simulink model "P3_model"  (R2025b)
settings: Solver=ode4  StartTime=0.0  StopTime=3  FixedStep=20e-6  RelTol=1e-3
model workspace (MATLAB code in the model file):
  | J = 0.01;  B = 0.10;                 % 참 플랜트
  | Jm = 0.01; Bm = 0.03;                % 공칭 모델
  | lam = 40;  Ts = 1e-3;  umax = 2;
  | beta = 0.37; phi = 0.05;             % phi = 0 이면 sgn
  | k = 1e-3;  rho = 0;  wc = 100;
  | adapt_on = 0; dob_on = 0;
  | dz = 0; vel_diff = 0; sigma_x = 0;   % 보너스용
  | P = struct('Jm',Jm,'Bm',Bm,'lam',lam,'Ts',Ts,'umax',umax, ...
  |            'beta',beta,'phi',phi,'k',k,'rho',rho,'wc',wc, ...
  |            'adapt_on',adapt_on,'dob_on',dob_on,'dz',dz,'vel_diff',vel_diff);
settings Model: Creator=Owner  LastModifiedBy=Owner

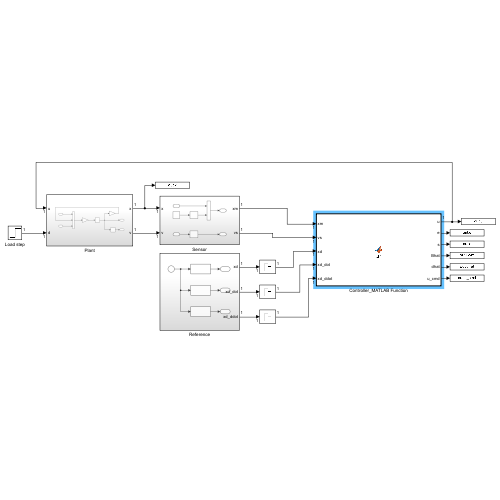
[thumbnail: Simulink's stored preview of the top-level diagram]
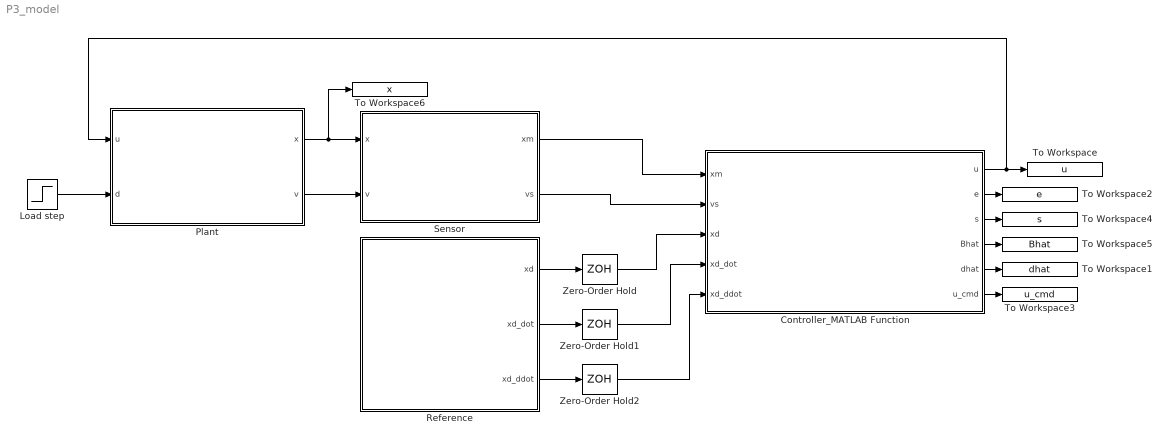
== system P3_model ==
  Controller_MATLAB Function : MATLAB Function  TreatAsAtomicUnit=on
  Load step : Step  Time=1.5  After=0.1  SampleTime=0
  Plant : Subsystem
  Reference : Subsystem
  Sensor : Subsystem
  To Workspace : ToWorkspace  VariableName=u  SaveFormat=Timeseries  SampleTime=-1
  To Workspace1 : ToWorkspace  VariableName=dhat  SaveFormat=Timeseries  SampleTime=-1
  To Workspace2 : ToWorkspace  VariableName=e  SaveFormat=Timeseries  SampleTime=-1
  To Workspace3 : ToWorkspace  VariableName=u_cmd  SaveFormat=Timeseries  SampleTime=-1
  To Workspace4 : ToWorkspace  VariableName=s  SaveFormat=Timeseries  SampleTime=-1
  To Workspace5 : ToWorkspace  VariableName=Bhat  SaveFormat=Timeseries  SampleTime=-1
  To Workspace6 : ToWorkspace  VariableName=x  SaveFormat=Timeseries  SampleTime=-1
  Zero-Order Hold : ZeroOrderHold  SampleTime=Ts
  Zero-Order Hold1 : ZeroOrderHold  SampleTime=Ts
  Zero-Order Hold2 : ZeroOrderHold  SampleTime=Ts
  wires:
  Load step/1 -> Plant/2(d)
  Sensor/1(xm) -> Controller_MATLAB Function/1(xm)
  Sensor/2(vs) -> Controller_MATLAB Function/2(vs)
  Reference/1(xd) -> Zero-Order Hold/1
  Reference/2(xd_dot) -> Zero-Order Hold1/1
  Reference/3(xd_ddot) -> Zero-Order Hold2/1
  Zero-Order Hold/1 -> Controller_MATLAB Function/3(xd)
  Zero-Order Hold1/1 -> Controller_MATLAB Function/4(xd_dot)
  Zero-Order Hold2/1 -> Controller_MATLAB Function/5(xd_ddot)
  Plant/1(x) -> To Workspace6/1, Sensor/1(x)
  Plant/2(v) -> Sensor/2(v)
  Controller_MATLAB Function/1(u) -> To Workspace/1, Plant/1(u)
  Controller_MATLAB Function/2(e) -> To Workspace2/1
  Controller_MATLAB Function/3(s) -> To Workspace4/1
  Controller_MATLAB Function/4(Bhat) -> To Workspace5/1
  Controller_MATLAB Function/5(dhat) -> To Workspace1/1
  Controller_MATLAB Function/6(u_cmd) -> To Workspace3/1

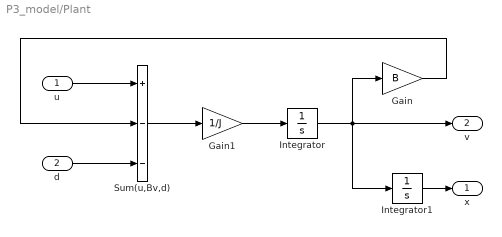
== system P3_model/Plant ==
  u : Inport
  d : Inport  Port=2
  Gain : Gain  Gain=B
  Gain1 : Gain  Gain=1/J
  Integrator : Integrator
  Integrator1 : Integrator
  Sum(u,Bv,d) : Sum  Inputs=+--
  x : Outport
  v : Outport  Port=2
  wires:
  Sum(u,Bv,d)/1 -> Gain1/1
  Gain1/1 -> Integrator/1
  Integrator/1 -> Gain/1, Integrator1/1, v/1
  u/1 -> Sum(u,Bv,d)/1
  d/1 -> Sum(u,Bv,d)/3
  Integrator1/1 -> x/1
  Gain/1 -> Sum(u,Bv,d)/2

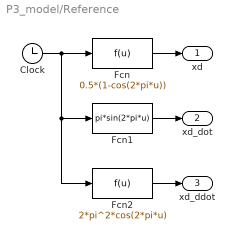
== system P3_model/Reference ==
  Clock : Clock
  Fcn : Fcn  Expr=0.5*(1-cos(2*pi*u))
  Fcn1 : Fcn  Expr=pi*sin(2*pi*u)
  Fcn2 : Fcn  Expr=2*pi^2*cos(2*pi*u)
  xd : Outport
  xd_dot : Outport  Port=2
  xd_ddot : Outport  Port=3
  wires:
  Clock/1 -> Fcn2/1, Fcn1/1, Fcn/1
  Fcn2/1 -> xd_ddot/1
  Fcn1/1 -> xd_dot/1
  Fcn/1 -> xd/1

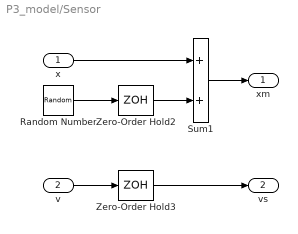
== system P3_model/Sensor ==
  x : Inport
  v : Inport  Port=2
  Random Number : RandomNumber  Variance=sigma_x^2  Seed=1  SampleTime=Ts
  Sum1 : Sum
  Zero-Order Hold2 : ZeroOrderHold  SampleTime=Ts
  Zero-Order Hold3 : ZeroOrderHold  SampleTime=Ts
  xm : Outport
  vs : Outport  Port=2
  wires:
  Random Number/1 -> Zero-Order Hold2/1
  Zero-Order Hold2/1 -> Sum1/2
  x/1 -> Sum1/1
  Sum1/1 -> xm/1
  v/1 -> Zero-Order Hold3/1
  Zero-Order Hold3/1 -> vs/1

== matlab function P3_model/Controller_MATLAB Function ==
  settings: updateMethod=DISCRETE  sampleTime=Ts
  data: xm input; u output; vs input; xd input; xd_dot input; xd_ddot input; e output; s output; Bhat output; dhat output; u_cmd output; P parameter
function [u, e, s, Bhat, dhat, u_cmd] = ctrl(xm, vs, xd, xd_dot, xd_ddot, P)
% ---- 출력 기본값 (모든 경로에서 정의되도록) ----
u = 0; e = 0; s = 0; Bhat = 0; dhat = 0; u_cmd = 0;

% ---- 상태 변수 ----
persistent ie Bh z xprev
if isempty(ie)
    ie = 0; Bh = P.Bm; z = 0; xprev = xm;
end

% ---- 속도: 측정값, 또는 위치 차분(보너스) ----
if P.vel_diff > 0.5
    vm = (xm - xprev)/P.Ts;
else
    vm = vs;
end
xprev = xm;

% ---- 슬라이딩 면 (e = xd - x) ----
e    = xd - xm;
de   = xd_dot - vm;
ie_t = ie + P.Ts*e;
s    = de + 2*P.lam*e + P.lam^2*ie_t;

% ---- 스위칭: phi = 0 이면 sgn, 아니면 sat ----
if P.phi == 0
    sw = sign(s);
else
    sw = min(max(s/P.phi, -1), 1);
end

% ---- 등가 제어 ----
if P.adapt_on > 0.5
    Bu = Bh;
else
    Bu = P.Bm;
end
ueq = P.Jm*xd_ddot + Bu*vm + P.Jm*(2*P.lam*de + P.lam^2*e);

% ---- DOB ----
dhat = P.dob_on*(z - P.Jm*P.wc*vm);

% ---- 제어 입력과 포화 ----
u_cmd = ueq + P.beta*sw + dhat;
u     = min(max(u_cmd, -P.umax), P.umax);

% ---- anti-windup: 포화 아닐 때만 적분 확정 ----
if abs(u_cmd) <= P.umax
    ie = ie_t;
end

% ---- 적응법칙 (누설 rho, 데드존 dz, clip [0, 0.5]) ----
if P.adapt_on > 0.5 && abs(s) >= P.dz
        Bh = Bh + P.Ts*P.k*(vm*sw/P.Jm - P.rho*(Bh - P.Bm));
    Bh = min(max(Bh, 0), 0.5);
end
Bhat = Bh;

% ---- DOB 상태 갱신 ----
z = z + P.Ts*P.wc*((u - P.Bm*vm + P.Jm*P.wc*vm) - z);
